simulink subsystem "GateDriver"  (R2025b)
settings: Solver=VariableStepAuto
model mask{DeadTime=DeadTime, DeadTimeSample=DeadTimeSample}
settings Model: Creator=kara  LastModifiedBy=Cheng
settings RTWCC: GPUComputeCapability=3.5

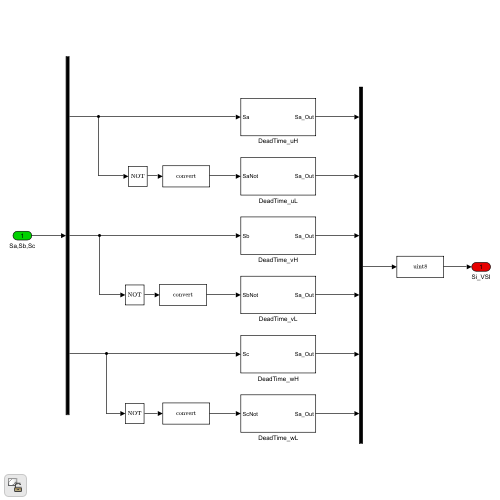
[thumbnail: Simulink's stored preview of the top-level diagram]
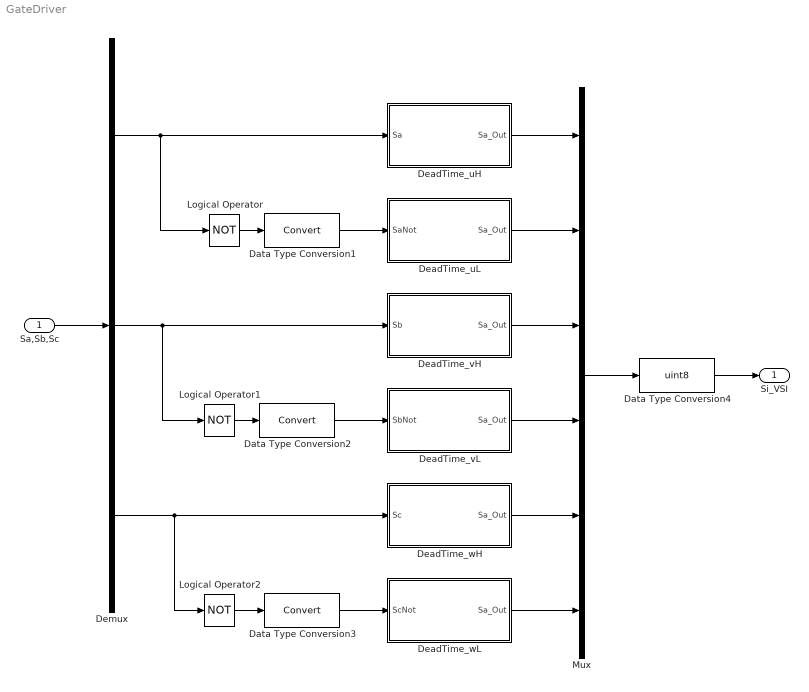
== system GateDriver ==
  Sa,Sb,Sc : Inport
  Data Type Conversion1 : DataTypeConversion  SaturateOnIntegerOverflow=off  RndMeth=Floor
  Data Type Conversion2 : DataTypeConversion  SaturateOnIntegerOverflow=off  RndMeth=Floor
  Data Type Conversion3 : DataTypeConversion  SaturateOnIntegerOverflow=off  RndMeth=Floor
  Data Type Conversion4 : DataTypeConversion  OutDataTypeStr=uint8  SaturateOnIntegerOverflow=off  RndMeth=Floor
  DeadTime_uH : Subsystem
  DeadTime_uL : Subsystem
  DeadTime_vH : Subsystem
  DeadTime_vL : Subsystem
  DeadTime_wH : Subsystem
  DeadTime_wL : Subsystem
  Demux : Demux  Outputs=3
  Logical Operator : Logic  Operator=NOT  AllPortsSameDT=off  OutDataTypeStr=boolean
  Logical Operator1 : Logic  Operator=NOT  AllPortsSameDT=off  OutDataTypeStr=boolean
  Logical Operator2 : Logic  Operator=NOT  AllPortsSameDT=off  OutDataTypeStr=boolean
  Mux : Mux  Inputs=6
  Si_VSI : Outport
  wires:
  DeadTime_wL/1(Sa_Out) -> Mux/6
  Data Type Conversion3/1 -> DeadTime_wL/1(ScNot)
  DeadTime_vL/1(Sa_Out) -> Mux/4
  Data Type Conversion2/1 -> DeadTime_vL/1(SbNot)
  DeadTime_vH/1(Sa_Out) -> Mux/3
  DeadTime_uL/1(Sa_Out) -> Mux/2
  Data Type Conversion1/1 -> DeadTime_uL/1(SaNot)
  Demux/1 -> DeadTime_uH/1(Sa), Logical Operator/1
  DeadTime_uH/1(Sa_Out) -> Mux/1
  Sa,Sb,Sc/1 -> Demux/1
  DeadTime_wH/1(Sa_Out) -> Mux/5
  Logical Operator2/1 -> Data Type Conversion3/1
  Demux/3 -> Logical Operator2/1, DeadTime_wH/1(Sc)
  Logical Operator1/1 -> Data Type Conversion2/1
  Demux/2 -> Logical Operator1/1, DeadTime_vH/1(Sb)
  Logical Operator/1 -> Data Type Conversion1/1
  Mux/1 -> Data Type Conversion4/1
  Data Type Conversion4/1 -> Si_VSI/1

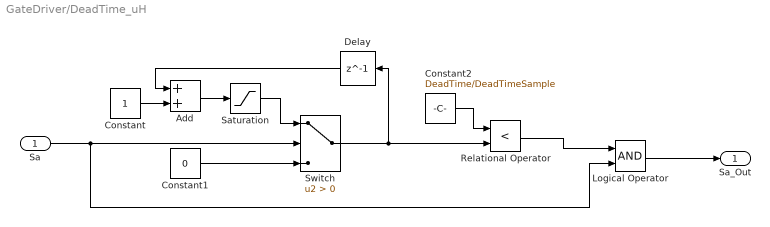
== system GateDriver/DeadTime_uH ==
  Sa : Inport
  Add : Sum
  Constant : Constant  OutDataTypeStr=uint8
  Constant1 : Constant  Value=0  OutDataTypeStr=uint8
  Constant2 : Constant  Value=DeadTime/DeadTimeSample  OutDataTypeStr=uint8
  Delay : Delay  DelayLength=1  InitialCondition=0
  Logical Operator : Logic  AllPortsSameDT=off  OutDataTypeStr=boolean
  Relational Operator : RelationalOperator  Operator=<  OutDataTypeStr=boolean  RndMeth=Simplest  InputSameDT=off
  Saturation : Saturate  UpperLimit=DeadTime/DeadTimeSample+1  LowerLimit=0
  Switch : Switch  Criteria=u2 > Threshold  OutDataTypeStr=uint8  SaturateOnIntegerOverflow=off  InputSameDT=off
  Sa_Out : Outport
  wires:
  Relational Operator/1 -> Logical Operator/1
  Constant2/1 -> Relational Operator/1
  Add/1 -> Saturation/1
  Constant/1 -> Add/2
  Delay/1 -> Add/1
  Switch/1 -> Delay/1, Relational Operator/2
  Sa/1 -> Switch/2, Logical Operator/2
  Logical Operator/1 -> Sa_Out/1
  Constant1/1 -> Switch/3
  Saturation/1 -> Switch/1

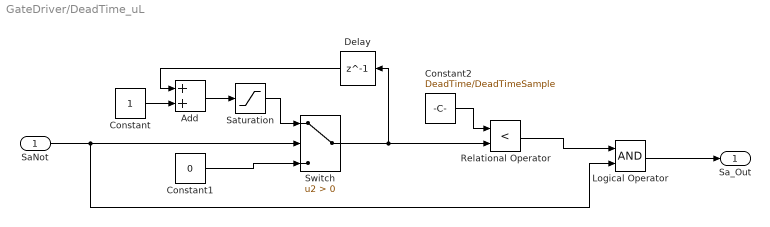
== system GateDriver/DeadTime_uL ==
  SaNot : Inport
  Add : Sum
  Constant : Constant  OutDataTypeStr=uint8
  Constant1 : Constant  Value=0  OutDataTypeStr=uint8
  Constant2 : Constant  Value=DeadTime/DeadTimeSample  OutDataTypeStr=uint8
  Delay : Delay  DelayLength=1  InitialCondition=0
  Logical Operator : Logic  AllPortsSameDT=off  OutDataTypeStr=boolean
  Relational Operator : RelationalOperator  Operator=<  OutDataTypeStr=boolean  RndMeth=Simplest  InputSameDT=off
  Saturation : Saturate  UpperLimit=DeadTime/DeadTimeSample+1  LowerLimit=0
  Switch : Switch  Criteria=u2 > Threshold  OutDataTypeStr=uint8  SaturateOnIntegerOverflow=off  InputSameDT=off
  Sa_Out : Outport
  wires:
  Logical Operator/1 -> Sa_Out/1
  SaNot/1 -> Logical Operator/2, Switch/2
  Switch/1 -> Relational Operator/2, Delay/1
  Delay/1 -> Add/1
  Constant/1 -> Add/2
  Add/1 -> Saturation/1
  Constant1/1 -> Switch/3
  Constant2/1 -> Relational Operator/1
  Relational Operator/1 -> Logical Operator/1
  Saturation/1 -> Switch/1

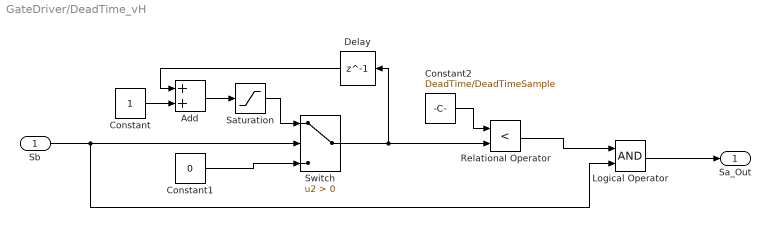
== system GateDriver/DeadTime_vH ==
  Sb : Inport
  Add : Sum
  Constant : Constant  OutDataTypeStr=uint8
  Constant1 : Constant  Value=0  OutDataTypeStr=uint8
  Constant2 : Constant  Value=DeadTime/DeadTimeSample  OutDataTypeStr=uint8
  Delay : Delay  DelayLength=1  InitialCondition=0
  Logical Operator : Logic  AllPortsSameDT=off  OutDataTypeStr=boolean
  Relational Operator : RelationalOperator  Operator=<  OutDataTypeStr=boolean  RndMeth=Simplest  InputSameDT=off
  Saturation : Saturate  UpperLimit=DeadTime/DeadTimeSample+1  LowerLimit=0
  Switch : Switch  Criteria=u2 > Threshold  OutDataTypeStr=uint8  SaturateOnIntegerOverflow=off  InputSameDT=off
  Sa_Out : Outport
  wires:
  Relational Operator/1 -> Logical Operator/1
  Constant2/1 -> Relational Operator/1
  Constant1/1 -> Switch/3
  Add/1 -> Saturation/1
  Constant/1 -> Add/2
  Delay/1 -> Add/1
  Switch/1 -> Delay/1, Relational Operator/2
  Sb/1 -> Switch/2, Logical Operator/2
  Logical Operator/1 -> Sa_Out/1
  Saturation/1 -> Switch/1

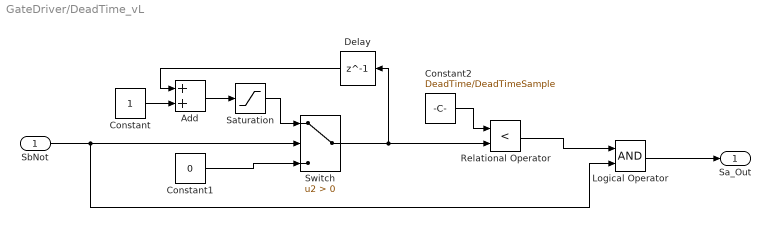
== system GateDriver/DeadTime_vL ==
  SbNot : Inport
  Add : Sum
  Constant : Constant  OutDataTypeStr=uint8
  Constant1 : Constant  Value=0  OutDataTypeStr=uint8
  Constant2 : Constant  Value=DeadTime/DeadTimeSample  OutDataTypeStr=uint8
  Delay : Delay  DelayLength=1  InitialCondition=0
  Logical Operator : Logic  AllPortsSameDT=off  OutDataTypeStr=boolean
  Relational Operator : RelationalOperator  Operator=<  OutDataTypeStr=boolean  RndMeth=Simplest  InputSameDT=off
  Saturation : Saturate  UpperLimit=DeadTime/DeadTimeSample+1  LowerLimit=0
  Switch : Switch  Criteria=u2 > Threshold  OutDataTypeStr=uint8  SaturateOnIntegerOverflow=off  InputSameDT=off
  Sa_Out : Outport
  wires:
  Logical Operator/1 -> Sa_Out/1
  SbNot/1 -> Logical Operator/2, Switch/2
  Switch/1 -> Relational Operator/2, Delay/1
  Delay/1 -> Add/1
  Constant/1 -> Add/2
  Add/1 -> Saturation/1
  Constant1/1 -> Switch/3
  Constant2/1 -> Relational Operator/1
  Relational Operator/1 -> Logical Operator/1
  Saturation/1 -> Switch/1

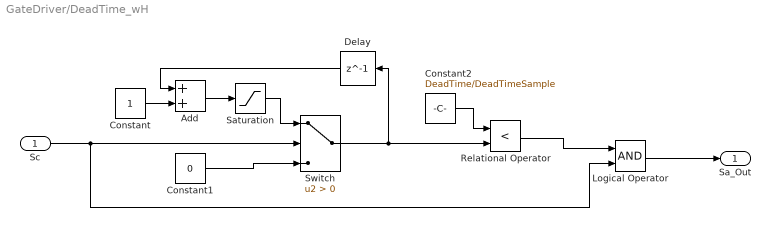
== system GateDriver/DeadTime_wH ==
  Sc : Inport
  Add : Sum
  Constant : Constant  OutDataTypeStr=uint8
  Constant1 : Constant  Value=0  OutDataTypeStr=uint8
  Constant2 : Constant  Value=DeadTime/DeadTimeSample  OutDataTypeStr=uint8
  Delay : Delay  DelayLength=1  InitialCondition=0
  Logical Operator : Logic  AllPortsSameDT=off  OutDataTypeStr=boolean
  Relational Operator : RelationalOperator  Operator=<  OutDataTypeStr=boolean  RndMeth=Simplest  InputSameDT=off
  Saturation : Saturate  UpperLimit=DeadTime/DeadTimeSample+1  LowerLimit=0
  Switch : Switch  Criteria=u2 > Threshold  OutDataTypeStr=uint8  SaturateOnIntegerOverflow=off  InputSameDT=off
  Sa_Out : Outport
  wires:
  Relational Operator/1 -> Logical Operator/1
  Constant2/1 -> Relational Operator/1
  Constant1/1 -> Switch/3
  Add/1 -> Saturation/1
  Constant/1 -> Add/2
  Delay/1 -> Add/1
  Switch/1 -> Delay/1, Relational Operator/2
  Sc/1 -> Switch/2, Logical Operator/2
  Logical Operator/1 -> Sa_Out/1
  Saturation/1 -> Switch/1

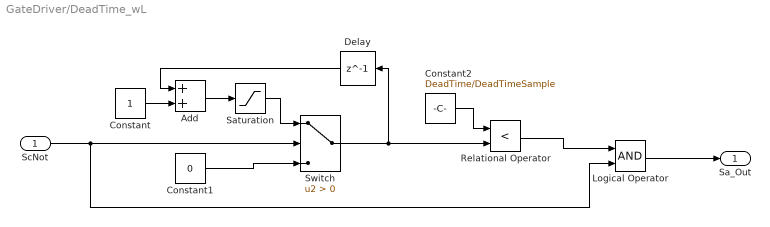
== system GateDriver/DeadTime_wL ==
  ScNot : Inport
  Add : Sum
  Constant : Constant  OutDataTypeStr=uint8
  Constant1 : Constant  Value=0  OutDataTypeStr=uint8
  Constant2 : Constant  Value=DeadTime/DeadTimeSample  OutDataTypeStr=uint8
  Delay : Delay  DelayLength=1  InitialCondition=0
  Logical Operator : Logic  AllPortsSameDT=off  OutDataTypeStr=boolean
  Relational Operator : RelationalOperator  Operator=<  OutDataTypeStr=boolean  RndMeth=Simplest  InputSameDT=off
  Saturation : Saturate  UpperLimit=DeadTime/DeadTimeSample+1  LowerLimit=0
  Switch : Switch  Criteria=u2 > Threshold  OutDataTypeStr=uint8  SaturateOnIntegerOverflow=off  InputSameDT=off
  Sa_Out : Outport
  wires:
  Logical Operator/1 -> Sa_Out/1
  ScNot/1 -> Logical Operator/2, Switch/2
  Switch/1 -> Relational Operator/2, Delay/1
  Delay/1 -> Add/1
  Constant/1 -> Add/2
  Add/1 -> Saturation/1
  Constant1/1 -> Switch/3
  Constant2/1 -> Relational Operator/1
  Relational Operator/1 -> Logical Operator/1
  Saturation/1 -> Switch/1
